simulink model "anesthesim"  (R2025b)
settings: Solver=ode15s  StartTime=0.0  StopTime=3600  MaxStep=Ts  RelTol=1e-4
undefined symbols (not defined in the file or in its folder): models, pHemo, Ts
settings Model: Creator=iza  LastModifiedBy=iza
settings DataIOCC: SaveOutput=off  SignalLogging=off  SaveTime=off

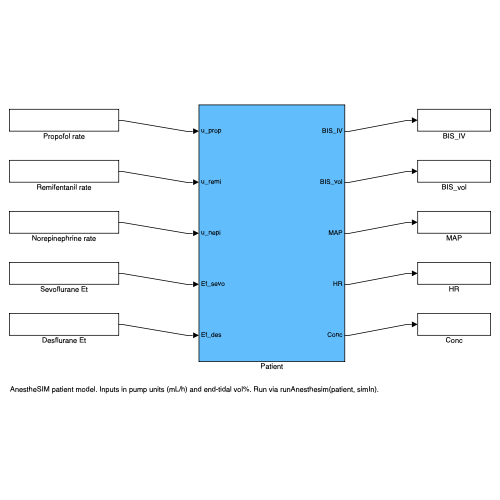
[thumbnail: Simulink's stored preview of the top-level diagram]
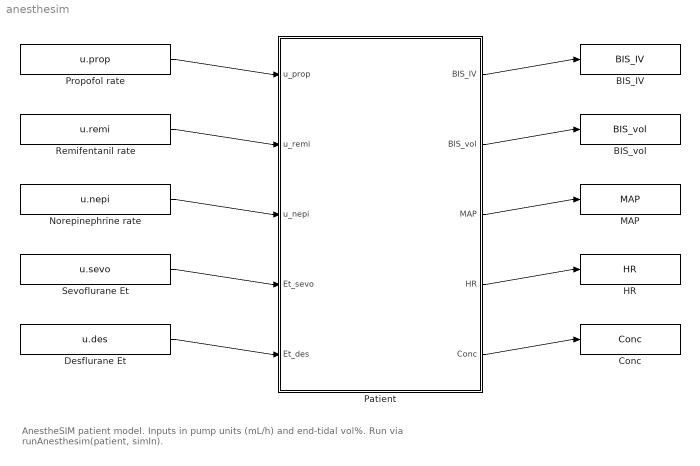
== system anesthesim ==
  note: AnestheSIM patient model. Inputs in pump units (mL/h) and end-tidal vol%. Run via runAnesthesim(patient, simIn).
  BIS_IV : ToWorkspace  VariableName=BIS_IV  SaveFormat=Timeseries  SampleTime=Ts
  BIS_vol : ToWorkspace  VariableName=BIS_vol  SaveFormat=Timeseries  SampleTime=Ts
  Conc : ToWorkspace  VariableName=Conc  SaveFormat=Timeseries  SampleTime=Ts
  Desflurane Et : FromWorkspace  VariableName=u.des  SampleTime=Ts  Interpolate=off  OutputAfterFinalValue=Holding final value
  HR : ToWorkspace  VariableName=HR  SaveFormat=Timeseries  SampleTime=Ts
  MAP : ToWorkspace  VariableName=MAP  SaveFormat=Timeseries  SampleTime=Ts
  Norepinephrine rate : FromWorkspace  VariableName=u.nepi  SampleTime=Ts  Interpolate=off  OutputAfterFinalValue=Holding final value
  Patient : Subsystem
  Propofol rate : FromWorkspace  VariableName=u.prop  SampleTime=Ts  Interpolate=off  OutputAfterFinalValue=Holding final value
  Remifentanil rate : FromWorkspace  VariableName=u.remi  SampleTime=Ts  Interpolate=off  OutputAfterFinalValue=Holding final value
  Sevoflurane Et : FromWorkspace  VariableName=u.sevo  SampleTime=Ts  Interpolate=off  OutputAfterFinalValue=Holding final value
  wires:
  Propofol rate/1 -> Patient/1(u_prop)
  Remifentanil rate/1 -> Patient/2(u_remi)
  Norepinephrine rate/1 -> Patient/3(u_nepi)
  Sevoflurane Et/1 -> Patient/4(Et_sevo)
  Desflurane Et/1 -> Patient/5(Et_des)
  Patient/1(BIS_IV) -> BIS_IV/1
  Patient/2(BIS_vol) -> BIS_vol/1
  Patient/3(MAP) -> MAP/1
  Patient/4(HR) -> HR/1
  Patient/5(Conc) -> Conc/1

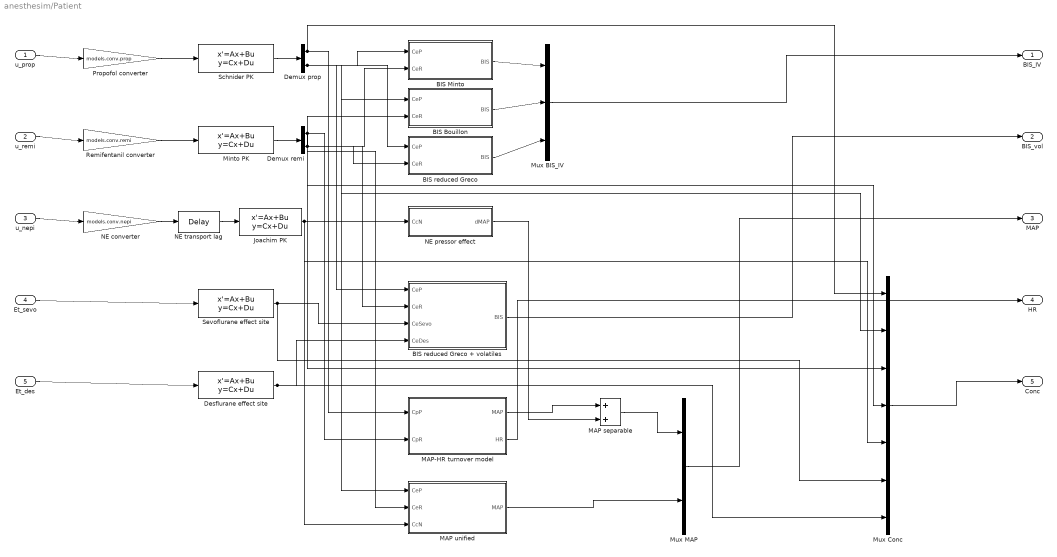
== system anesthesim/Patient ==
  u_prop : Inport  Description=propofol pump rate [mL/h]
  u_remi : Inport  Description=remifentanil pump rate [mL/h]  Port=2
  u_nepi : Inport  Description=norepinephrine pump rate [mL/h]  Port=3
  Et_sevo : Inport  Description=end-tidal sevoflurane [vol%]  Port=4
  Et_des : Inport  Description=end-tidal desflurane [vol%]  Port=5
  BIS Bouillon : MATLAB Function  TreatAsAtomicUnit=on
  BIS Minto : MATLAB Function  TreatAsAtomicUnit=on
  BIS reduced Greco : MATLAB Function  TreatAsAtomicUnit=on
  BIS reduced Greco + volatiles : MATLAB Function  TreatAsAtomicUnit=on
  Demux prop : Demux  Outputs=2
  Demux remi : Demux  Outputs=2
  Desflurane effect site : StateSpace  A=models.des.A  B=models.des.B  C=models.des.C  D=models.des.D  InitialCondition=0
  Joachim PK : StateSpace  A=models.nepi.A  B=models.nepi.B  C=models.nepi.C  D=models.nepi.D  InitialCondition=0
  MAP separable : Sum
  MAP unified : MATLAB Function  TreatAsAtomicUnit=on
  MAP-HR turnover model : Subsystem
  Minto PK : StateSpace  A=models.remi.A  B=models.remi.B  C=models.remi.C  D=models.remi.D  InitialCondition=0
  Mux BIS_IV : Mux  Inputs=3
  Mux Conc : Mux  Inputs=7
  Mux MAP : Mux  Inputs=2
  NE converter : Gain  Gain=models.conv.nepi
  NE pressor effect : MATLAB Function  TreatAsAtomicUnit=on
  NE transport lag : TransportDelay  DelayTime=models.nepi.Tlag  BufferSize=16384
  Propofol converter : Gain  Gain=models.conv.prop
  Remifentanil converter : Gain  Gain=models.conv.remi
  Schnider PK : StateSpace  A=models.prop.A  B=models.prop.B  C=models.prop.C  D=models.prop.D  InitialCondition=0
  Sevoflurane effect site : StateSpace  A=models.sevo.A  B=models.sevo.B  C=models.sevo.C  D=models.sevo.D  InitialCondition=0
  BIS_IV : Outport
  BIS_vol : Outport  Port=2
  MAP : Outport  Port=3
  HR : Outport  Port=4
  Conc : Outport  Port=5
  wires:
  u_prop/1 -> Propofol converter/1
  Propofol converter/1 -> Schnider PK/1
  Schnider PK/1 -> Demux prop/1
  u_remi/1 -> Remifentanil converter/1
  Remifentanil converter/1 -> Minto PK/1
  Minto PK/1 -> Demux remi/1
  u_nepi/1 -> NE converter/1
  NE converter/1 -> NE transport lag/1
  NE transport lag/1 -> Joachim PK/1
  Et_sevo/1 -> Sevoflurane effect site/1
  Et_des/1 -> Desflurane effect site/1
  Demux prop/2 -> BIS Minto/1(CeP), BIS Bouillon/1(CeP), BIS reduced Greco/1(CeP), BIS reduced Greco + volatiles/1(CeP), MAP unified/1(CeP), Mux Conc/2
  Demux remi/2 -> BIS Minto/2(CeR), BIS Bouillon/2(CeR), BIS reduced Greco/2(CeR), BIS reduced Greco + volatiles/2(CeR), MAP unified/2(CeR), Mux Conc/4
  BIS Minto/1(BIS) -> Mux BIS_IV/1
  BIS Bouillon/1(BIS) -> Mux BIS_IV/2
  BIS reduced Greco/1(BIS) -> Mux BIS_IV/3
  Mux BIS_IV/1 -> BIS_IV/1
  Sevoflurane effect site/1 -> BIS reduced Greco + volatiles/3(CeSevo), Mux Conc/6
  Desflurane effect site/1 -> BIS reduced Greco + volatiles/4(CeDes), Mux Conc/7
  BIS reduced Greco + volatiles/1(BIS) -> BIS_vol/1
  Demux prop/1 -> MAP-HR turnover model/1(CpP), Mux Conc/1
  Demux remi/1 -> MAP-HR turnover model/2(CpR), Mux Conc/3
  Joachim PK/1 -> NE pressor effect/1(CcN), MAP unified/3(CcN), Mux Conc/5
  MAP-HR turnover model/1(MAP) -> MAP separable/1
  NE pressor effect/1(dMAP) -> MAP separable/2
  MAP separable/1 -> Mux MAP/1
  MAP unified/1(MAP) -> Mux MAP/2
  Mux MAP/1 -> MAP/1
  MAP-HR turnover model/2(HR) -> HR/1
  Mux Conc/1 -> Conc/1

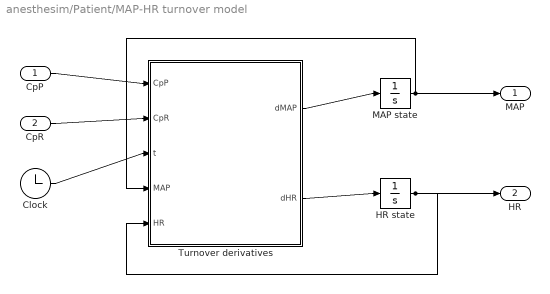
== system anesthesim/Patient/MAP-HR turnover model ==
  CpP : Inport
  CpR : Inport  Port=2
  Clock : Clock
  HR state : Integrator  InitialCondition=pHemo.HR0
  MAP state : Integrator  InitialCondition=pHemo.MAP0
  Turnover derivatives : MATLAB Function  TreatAsAtomicUnit=on
  MAP : Outport
  HR : Outport  Port=2
  wires:
  CpP/1 -> Turnover derivatives/1(CpP)
  CpR/1 -> Turnover derivatives/2(CpR)
  Clock/1 -> Turnover derivatives/3(t)
  Turnover derivatives/1(dMAP) -> MAP state/1
  Turnover derivatives/2(dHR) -> HR state/1
  MAP state/1 -> MAP/1, Turnover derivatives/4(MAP)
  HR state/1 -> HR/1, Turnover derivatives/5(HR)

== matlab function anesthesim/Patient/BIS Bouillon ==
  data: CeP input; BIS output; CeR input; pBisBouillon parameter
function BIS = fcn(CeP, CeR, pBisBouillon)
%#codegen
BIS = bisBouillon(CeP, CeR, pBisBouillon);
end

== matlab function anesthesim/Patient/BIS Minto ==
  data: CeP input; BIS output; CeR input; pBisMinto parameter
function BIS = fcn(CeP, CeR, pBisMinto)
%#codegen
BIS = bisMinto(CeP, CeR, pBisMinto);
end

== matlab function anesthesim/Patient/BIS reduced Greco ==
  data: CeP input; BIS output; CeR input; pBisGreco parameter
function BIS = fcn(CeP, CeR, pBisGreco)
%#codegen
BIS = bisGreco(CeP, CeR, pBisGreco);
end

== matlab function anesthesim/Patient/BIS reduced Greco + volatiles ==
  data: CeP input; BIS output; CeR input; CeSevo input; CeDes input; pBisVolatile parameter
function BIS = fcn(CeP, CeR, CeSevo, CeDes, pBisVolatile)
%#codegen
BIS = bisGrecoVolatile(CeP, CeR, CeSevo, CeDes, pBisVolatile);
end

== matlab function anesthesim/Patient/MAP-HR turnover model/Turnover derivatives ==
  data: CpP input; dMAP output; CpR input; t input; MAP input; HR input; dHR output; pHemo parameter
function [dMAP, dHR] = fcn(CpP, CpR, t, MAP, HR, pHemo)
%#codegen
[dMAP, dHR] = hemodynamicTurnover(CpP, CpR, t, MAP, HR, pHemo);
end

== matlab function anesthesim/Patient/NE pressor effect ==
  data: CcN input; dMAP output; pNE parameter
function dMAP = fcn(CcN, pNE)
%#codegen
dMAP = norepinephrineEffect(CcN, pNE);
end

== matlab function anesthesim/Patient/MAP unified ==
  data: CeP input; MAP output; CeR input; CcN input; pMapUnified parameter
function MAP = fcn(CeP, CeR, CcN, pMapUnified)
%#codegen
MAP = mapUnified(CeP, CeR, CcN, pMapUnified);
end
